simulink model "Intro_LQR_Demo"  (R2025b)
settings: Solver=ode45  StartTime=0.0  StopTime=15  MaxStep=0.01  RelTol=1e-6  AbsTol=1e-8
InitFcn:
  | evalin(get_param(bdroot,'ModelWorkspace'),'assert(m>0 && g>0 && a>0 && I>0, ''Physical parameters must be positive.''); A = zeros(6); A(1,2)=1; A(2,5)=-g; A(3,4)=1; A(5,6)=1; B = zeros(6,2); B(2,2)=-g; B(4,1)=1/m; B(6,2)=-a*m*g/I; assert(rank(ctrb(A,B))==6, ''Hover model must be controllable.''); [K,S,closedLoopPoles] = lqr(A,B,Q,R); Uhover = [m*g;0]; assert(F_max>m*g && phi_max>0, ''Limits must allow hover and tilt correction.''); assert(numel(Xref)==6 && all(Xref([2 4 5 6])==0), ''Use a stationary upright reference.'');');
model workspace (MAT data in the model file):
  A = [0  1  0  0  0  0; 0  0  0  0  -9.81  0; 0  0  0  1  0  0; 0  0  0  0  0  0; 0  0  0  0  0  1; 0  0  0  0  0  0]
  B = [0  0; 0  -9.81; 0  0; 1  0; 0  0; 0  -9.81]
  F_max = 20
  I = 1
  K = [1.9545198688e-15  3.79814540621e-15  6.32455532034  4.20108446007  -1.997851147e-14  -9.59385557703e-15; 1  2.25228622108  -7.47331063035e-16  2.83401229821e-17  -19.9770507522  -7.71753275013]
  Q = [1  0  0  0  0  0; 0  1  0  0  0  0; 0  0  4  0  0  0; 0  0  0  0.5  0  0; 0  0  0  0  100  0; 0  0  0  0  0  25]
  R = [0.1  0; 0  1]
  S = [2.25228622108  2.03639661083  -3.74540196132e-16  1.56459587931e-16  -7.71753275013  -2.13833341001; 2.03639661083  3.79984744106  -2.96574577286e-16  3.18767359992e-16  -15.2437592638  -4.02943828928; -3.74540196132e-16  -2.96574577286e-16  2.65699910731  0.632455532034  2.33881715594e-15  4.55450128469e-16; 1.56459587931e-16  3.18767359992e-16  0.632455532034  0.420108446007  -1.30614346581e-15  -2.28453365067e-16; -7.71753275013  -15.2437592638  2.33881715594e-15  -1.30614346581e-15  114.644753813  17.2801558746; -2.13833341001  -4.02943828928  4.55450128469e-16  -2.28453365067e-16  17.2801558746  4.81613887543]
  Ts_noise = 0.01
  Uhover = [9.81; 0]
  X0 = [2; 0; 0; 0; 0.03; 0]
  Xref = [3; 0; 30; 0; 0; 0]
  a = 1
  closedLoopPoles = [-0.856099419086+0.516176821697i; -0.856099419086-0.516176821697i; -1.92695064432+0i; -2.10054223004+1.38285127912i; -2.10054223004-1.38285127912i; -49.9749189675+0i]
  g = 9.81
  m = 1
  phi_max = 0.17
  sigma = [0.03; 0.06; 0.03; 0.06; 0.006; 0.009]
libraries: simulink x1
settings Model: Creator=cmax0  LastModifiedBy=cmax0

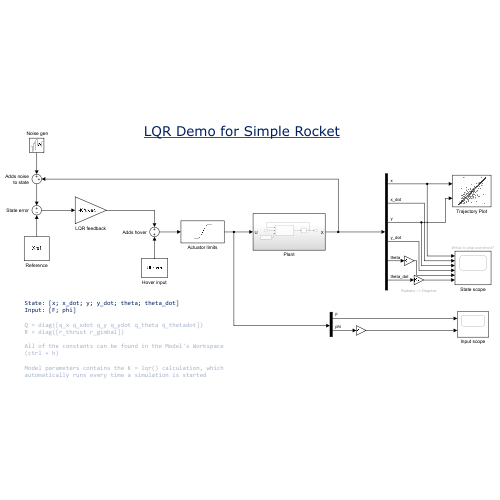
[thumbnail: Simulink's stored preview of the top-level diagram]
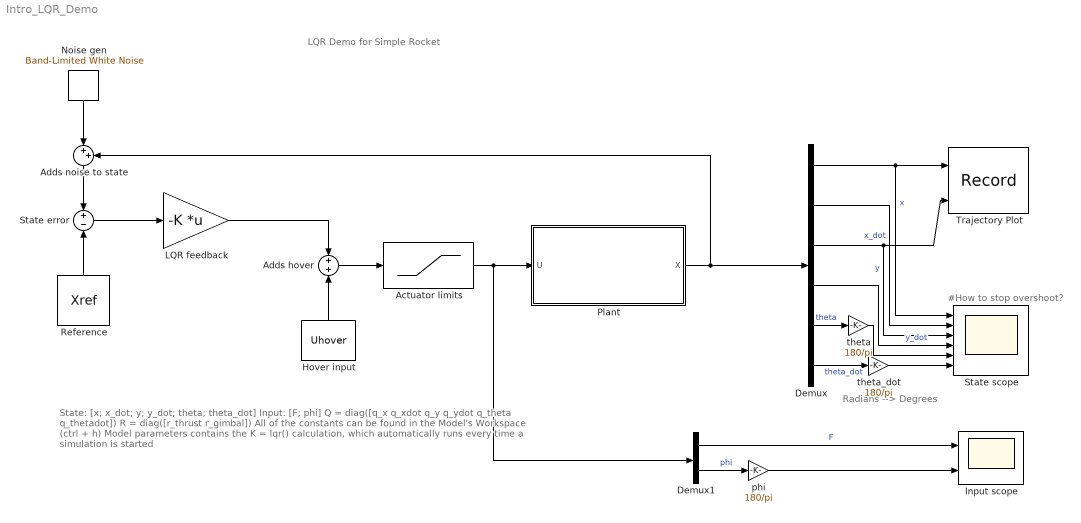
== system Intro_LQR_Demo ==
  note: #How to stop overshoot?
  note: LQR Demo for Simple Rocket
  note: State: [x; x_dot; y; y_dot; theta; theta_dot]
      | Input: [F; phi]
      |
      | Q = diag([q_x q_xdot q_y q_ydot q_theta q_thetadot])
      | R = diag([r_thrust r_gimbal])
      |
      | All of the constants can be found in the Model's Workspace (ctrl + h)
      |
      | Model parameters contains the K = lqr() calculation, which automatically runs every time a simulation is started
  note: Radians --> Degrees
  " Noise gen" : simulink/Sources/Band-Limited White Noise  Cov=sigma.^2 * Ts_noise  Ts=Ts_noise  seed=[11;22;33;44;55;66]
  Actuator limits : Saturate  UpperLimit=[F_max;phi_max]  LowerLimit=[0;-phi_max]
  Adds hover : Sum
  Adds noise to state : Sum  Inputs=|++
  Demux : Demux  Outputs=6
  Demux1 : Demux  Outputs=2
  Hover input : Constant  Value=Uhover
  Input scope : Scope  NumInputPorts=2
      settings: ActiveDisplayYMinimum=-9.207816529611673  ActiveDisplayYMaximum=33.207701324124656
  LQR feedback : Gain  Gain=-K  Multiplication=Matrix(K*u) (u vector)
  Plant : Subsystem
  Reference : Constant  Value=Xref
  State error : Sum  Inputs=+-
  State scope : Scope  NumInputPorts=6
      settings: ActiveDisplayYMinimum=-10.933064638251871  ActiveDisplayYMaximum=41.229990783143791
  Trajectory Plot : Record  NumPorts=2.0  FileSettingsInternal="{\"entries\":[{\"content\":{\"excelSettings\":{\"content\":{},\"type\":\"Streamout.ExcelSettings\"},\"parquetSettings\":{\"content\":{},\"type\":\"Streamout.ParquetSettings\"}},\"type\":\"Streamout.FileSettingStorage\",\"uuid\":\"\"}],\"packageUris\":[\"http:\\/\\/schema.mathworks.com\\/mf0\\/streamout_blocks\\/R2020a\"],\"version\":\"1.0\"}"  FrameSettings=[0, 0]  Layout=[1 1]  SignalsInternal="{\"entries\":[{\"content\":{\"signals\":[{\"content\":{\"blockPath\":[],\"dimensions\":[1,1],\"domain\":\"\",\"lineColor\":\"#a2142f\",\"plots\":[ 1 ],\"port\":1,\"sid\":[\"\"],\"signalID\":1,\"signalName\":\"x\"},\"type\":\"RecordBlkView.Signal\",\"uuid\":\"\"},{\"content\":{\"blockPath\":[],\"dimensions\":[1,1],\"domain\":\"\",\"lineColor\":\"#139fff\",\"plots\":[ 1 ],\"port\":2,\"sid\":[\"\"],\"signalID\":2,\"signalName\":\"y\"},\"type\":\"RecordBlkView.Signal\",\"uuid\":\"\"}]},\"type\":\"RecordBlkView.InputSignals\",\"uuid\":\"\"}],\"packageUris\":[\"http:\\/\\/schema.mathworks.com\\/mf0\\/streamout_blocks\\/R2020a\"],\"version\":\"1.0\"}"  VisualizationBindings="{\"xyplotplugin\":{\"info\":[{\"series\":[{\"bindingParametersList\":[{\"parameter\":\"X-Axis\",\"signalID\":1,\"signalName\":\"x\"},{\"parameter\":\"Y-Axis\",\"signalID\":2,\"signalName\":\"y\"}],\"seriesID\":0}],\"subplotID\":1}]}}"  CompatibilityTag=XY
  phi : Gain  Gain=180/pi
  theta : Gain  Gain=180/pi
  theta_dot : Gain  Gain=180/pi
  wires:
  Plant/1(X) -> Demux/1, Adds noise to state/2
  State error/1 -> LQR feedback/1
  LQR feedback/1 -> Adds hover/1
  Hover input/1 -> Adds hover/2
  Adds hover/1 -> Actuator limits/1
  Actuator limits/1 -> Demux1/1, Plant/1(U)
  Reference/1 -> State error/2
  Adds noise to state/1 -> State error/1
  " Noise gen"/1 -> Adds noise to state/1
  Demux/1 -> Trajectory Plot/1, State scope/1  "x"
  Demux/2 -> State scope/2  "x_dot"
  Demux/3 -> State scope/3, Trajectory Plot/2  "y"
  Demux/5 -> theta/1  "theta"
  Demux/6 -> theta_dot/1  "theta_dot"
  Demux/4 -> State scope/4  "y_dot"
  Demux1/1 -> Input scope/1  "F"
  Demux1/2 -> phi/1  "phi"
  theta/1 -> State scope/5
  theta_dot/1 -> State scope/6
  phi/1 -> Input scope/2

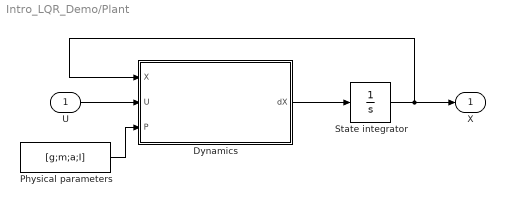
== system Intro_LQR_Demo/Plant ==
  U : Inport
  Dynamics : MATLAB Function  TreatAsAtomicUnit=on
  Physical parameters : Constant  Value=[g;m;a;I]
  State integrator : Integrator  InitialCondition=X0
  X : Outport
  wires:
  State integrator/1 -> Dynamics/1(X), X/1
  U/1 -> Dynamics/2(U)
  Physical parameters/1 -> Dynamics/3(P)
  Dynamics/1(dX) -> State integrator/1

== matlab function Intro_LQR_Demo/Plant/Dynamics ==
  data: X input size=[6 1]; dX output size=[6 1]; U input size=[2 1]; P input size=[4 1]
function dX = rocketDynamics(X, U, P)

% State: [x; x_dot; y; y_dot; theta; theta_dot]
% Input: [F; phi], Parameters: [g; m; a; I]

g = P(1); m = P(2); a = P(3); I = P(4);
theta = X(5); F = U(1); phi = U(2);

x_ddot = -F/m * sin(theta + phi);
y_ddot = -g + F/m * cos(theta + phi);
theta_ddot = -a * F * sin(phi) / I;

dX = [X(2); x_ddot; X(4); y_ddot; X(6); theta_ddot];
end
